simulink model "PSO_BON"  (R2019b)
settings: Solver=VariableStepAuto  StartTime=0.0  StopTime=0.2  RelTol=1e-5
undefined symbols (not defined in the file): sigbuilder_block
libraries: powerlib x164, re_lib x96, powerlib_meascontrol x9
(part 3 of 6)

== system PSO_BON/InCond1/Panel Surya/Subsystem12 ==
  In1 : Inport
  In2 : Inport  Port=2
  Diode1 : powerlib/Power Electronics/Diode  Ron=0.001  Lon=0  Vf=0.7  IC=0  UseSnubber=off  Rs=1e5*inf  Cs=inf  Measurements=off
      settings: SourceProductName=Simscape Electrical
  PV Module 5 : re_lib/Solar/PV Array  Npar=1  Nser=1  PlotType=array @ 25 deg.C & specified irradiances  S_vec="[ 1000  700  100 200]"  Temp_C_vec="[ 45 25  ]"  ModuleName=User-defined  PlotWhenSelected=off  Pm=21.837  Ncell=72  Voc=5.425  Isc=5.34  Vm=4.35  Im=5.02  beta_Voc_pc=-0.37501  alpha_Isc_pc=0.075  beta_Voc=-0.020344  alpha_Isc=0.004005  IL=5.3624  I0=3.052e-10  nI=0.12439  Rsh=79.3172  Rs=0.081018  BAL=off  Tc=1e-6  Tfilter=5e-5
      settings: SourceProductName=Simscape Electrical
  + : PMIOPort  Side=Right
  - : PMIOPort  Port=2  Side=Right
  wires:
  In1/1 -> PV Module 5/1
  In2/1 -> PV Module 5/2
  connections:
  Diode1/LConn1 -- -/RConn1 -- PV Module 5/RConn2
  +/RConn1 -- PV Module 5/RConn1 -- Diode1/RConn1

== system PSO_BON/InCond1/Panel Surya/Subsystem13 ==
  Gain{,1..3} (4 alike) : Gain  Gain=1000
  Signal Builder : Subsystem  Tag=STV Subsys  LoadFcn=sigbuilder_block('load');  StartFcn=sigbuilder_block('start');  StopFcn=sigbuilder_block('stop');  ClipboardFcn=sigbuilder_block('clipboard');  mask(Sigbuilder block){tuvar=[0:10]}
      mask help: Simulink:masks:SigbuilderBlock_MD
      mask init:
      | if ~strcmp(get_param(bdroot(gcbh),'SimulationStatus'),'stopped') tuvar = sigbuilder_block('maskInit'); end
      settings: CopyFcn=sigbuilder_block('copy');  DeleteFcn=sigbuilder_block('delete');  ModelCloseFcn=sigbuilder_block('modelClose');  PreSaveFcn=sigbuilder_block('preSave');  PauseFcn=sigbuilder_block('pause');  ContinueFcn=sigbuilder_block('continue');  NameChangeFcn=sigbuilder_block('namechange');  OpenFcn=sigbuilder_block('open',[0.75 36.75 510.75 475.5 ]);  CloseFcn=sigbuilder_block('close');
      mask Display: plot(0, 0, 100, 100,[2, 2, 32, 32, 2], [68, 8, 8, 68, 68],[32, 2], [38, 38], [32, 19, 2],[53, 60, 44], [32, 17, 17, 2],[16, 16, 31, 31]);txt = getActiveGroup(gcbh);text(2, 100, txt,'verticalAlignment', 'top');
  Out1 : Outport
  Out2 : Outport  Port=2
  Out3 : Outport  Port=3
  Out4 : Outport  Port=4
  wires:
  Gain/1 -> Out1/1
  Signal Builder/1(Signal 2) -> Gain/1
  Gain1/1 -> Out2/1
  Signal Builder/2(Signal 1) -> Gain1/1
  Gain2/1 -> Out3/1
  Signal Builder/3(Signal 3) -> Gain2/1
  Gain3/1 -> Out4/1
  Signal Builder/4(Signal 4) -> Gain3/1

== system PSO_BON/InCond1/Panel Surya/Subsystem17 ==
  In1 : Inport
  In2 : Inport  Port=2
  Diode1 : powerlib/Power Electronics/Diode  Ron=0.001  Lon=0  Vf=0.7  IC=0  UseSnubber=off  Rs=1e5*inf  Cs=inf  Measurements=off
      settings: SourceProductName=Simscape Electrical
  PV Module 5 : re_lib/Solar/PV Array  Npar=1  Nser=1  PlotType=array @ 25 deg.C & specified irradiances  S_vec="[ 1000  700  100 200]"  Temp_C_vec="[ 45 25  ]"  ModuleName=User-defined  PlotWhenSelected=off  Pm=21.837  Ncell=72  Voc=5.425  Isc=5.34  Vm=4.35  Im=5.02  beta_Voc_pc=-0.37501  alpha_Isc_pc=0.075  beta_Voc=-0.020344  alpha_Isc=0.004005  IL=5.3624  I0=3.052e-10  nI=0.12439  Rsh=79.3172  Rs=0.081018  BAL=off  Tc=1e-6  Tfilter=5e-5
      settings: SourceProductName=Simscape Electrical
  + : PMIOPort  Side=Right
  - : PMIOPort  Port=2  Side=Right
  wires:
  In2/1 -> PV Module 5/2
  In1/1 -> PV Module 5/1
  connections:
  Diode1/RConn1 -- PV Module 5/RConn1 -- +/RConn1
  PV Module 5/RConn2 -- -/RConn1 -- Diode1/LConn1

== system PSO_BON/InCond1/Panel Surya/Subsystem18 ==
  In1 : Inport
  In2 : Inport  Port=2
  Diode1 : powerlib/Power Electronics/Diode  Ron=0.001  Lon=0  Vf=0.7  IC=0  UseSnubber=off  Rs=1e5*inf  Cs=inf  Measurements=off
      settings: SourceProductName=Simscape Electrical
  PV Module 5 : re_lib/Solar/PV Array  Npar=1  Nser=1  PlotType=array @ 25 deg.C & specified irradiances  S_vec="[ 1000  700  100 200]"  Temp_C_vec="[ 45 25  ]"  ModuleName=User-defined  PlotWhenSelected=off  Pm=21.837  Ncell=72  Voc=5.425  Isc=5.34  Vm=4.35  Im=5.02  beta_Voc_pc=-0.37501  alpha_Isc_pc=0.075  beta_Voc=-0.020344  alpha_Isc=0.004005  IL=5.3624  I0=3.052e-10  nI=0.12439  Rsh=79.3172  Rs=0.081018  BAL=off  Tc=1e-6  Tfilter=5e-5
      settings: SourceProductName=Simscape Electrical
  + : PMIOPort  Side=Right
  - : PMIOPort  Port=2  Side=Right
  wires:
  In1/1 -> PV Module 5/1
  In2/1 -> PV Module 5/2
  connections:
  Diode1/LConn1 -- -/RConn1 -- PV Module 5/RConn2
  +/RConn1 -- PV Module 5/RConn1 -- Diode1/RConn1

== system PSO_BON/InCond1/Panel Surya/Subsystem19 ==
  In1 : Inport
  In2 : Inport  Port=2
  Diode1 : powerlib/Power Electronics/Diode  Ron=0.001  Lon=0  Vf=0.7  IC=0  UseSnubber=off  Rs=1e5*inf  Cs=inf  Measurements=off
      settings: SourceProductName=Simscape Electrical
  PV Module 5 : re_lib/Solar/PV Array  Npar=1  Nser=1  PlotType=array @ 25 deg.C & specified irradiances  S_vec="[ 1000  700  100 200]"  Temp_C_vec="[ 45 25  ]"  ModuleName=User-defined  PlotWhenSelected=off  Pm=21.837  Ncell=72  Voc=5.425  Isc=5.34  Vm=4.35  Im=5.02  beta_Voc_pc=-0.37501  alpha_Isc_pc=0.075  beta_Voc=-0.020344  alpha_Isc=0.004005  IL=5.3624  I0=3.052e-10  nI=0.12439  Rsh=79.3172  Rs=0.081018  BAL=off  Tc=1e-6  Tfilter=5e-5
      settings: SourceProductName=Simscape Electrical
  + : PMIOPort  Side=Right
  - : PMIOPort  Port=2  Side=Right
  wires:
  In2/1 -> PV Module 5/2
  In1/1 -> PV Module 5/1
  connections:
  Diode1/RConn1 -- PV Module 5/RConn1 -- +/RConn1
  PV Module 5/RConn2 -- -/RConn1 -- Diode1/LConn1

== system PSO_BON/InCond1/Panel Surya/Subsystem2 ==
  In1 : Inport
  In2 : Inport  Port=2
  Diode1 : powerlib/Power Electronics/Diode  Ron=0.001  Lon=0  Vf=0.7  IC=0  UseSnubber=off  Rs=1e5*inf  Cs=inf  Measurements=off
      settings: SourceProductName=Simscape Electrical
  PV Module 5 : re_lib/Solar/PV Array  Npar=1  Nser=1  PlotType=one module @ 25 deg.C & specified irradiances  S_vec="[ 1000  800  100 200]"  Temp_C_vec="[ 45 25  ]"  ModuleName=SunPower SPR-315E-WHT-D  PlotWhenSelected=off  Pm=315.072  Ncell=96  Voc=64.6  Isc=6.14  Vm=54.7  Im=5.76  beta_Voc_pc=-0.27269  alpha_Isc_pc=0.061694  beta_Voc=-0.17616  alpha_Isc=0.003788  IL=6.1461  I0=6.5043e-12  nI=0.9507  Rsh=430.0559  Rs=0.43042  BAL=off  Tc=1e-6  Tfilter=5e-5
      settings: SourceProductName=Simscape Electrical
  + : PMIOPort  Side=Right
  - : PMIOPort  Port=2  Side=Right
  wires:
  In1/1 -> PV Module 5/1
  In2/1 -> PV Module 5/2
  connections:
  Diode1/LConn1 -- -/RConn1 -- PV Module 5/RConn2
  +/RConn1 -- PV Module 5/RConn1 -- Diode1/RConn1

== system PSO_BON/InCond1/Panel Surya/Subsystem3 ==
  In1 : Inport
  In2 : Inport  Port=2
  Diode1 : powerlib/Power Electronics/Diode  Ron=0.001  Lon=0  Vf=0.7  IC=0  UseSnubber=off  Rs=1e5*inf  Cs=inf  Measurements=off
      settings: SourceProductName=Simscape Electrical
  PV Module 5 : re_lib/Solar/PV Array  Npar=1  Nser=1  PlotType=one module @ 25 deg.C & specified irradiances  S_vec="[ 1000  800  100 200]"  Temp_C_vec="[ 45 25  ]"  ModuleName=SunPower SPR-315E-WHT-D  PlotWhenSelected=off  Pm=315.072  Ncell=96  Voc=64.6  Isc=6.14  Vm=54.7  Im=5.76  beta_Voc_pc=-0.27269  alpha_Isc_pc=0.061694  beta_Voc=-0.17616  alpha_Isc=0.003788  IL=6.1461  I0=6.5043e-12  nI=0.9507  Rsh=430.0559  Rs=0.43042  BAL=off  Tc=1e-6  Tfilter=5e-5
      settings: SourceProductName=Simscape Electrical
  + : PMIOPort  Side=Right
  - : PMIOPort  Port=2  Side=Right
  wires:
  In2/1 -> PV Module 5/2
  In1/1 -> PV Module 5/1
  connections:
  Diode1/RConn1 -- PV Module 5/RConn1 -- +/RConn1
  PV Module 5/RConn2 -- -/RConn1 -- Diode1/LConn1

== system PSO_BON/InCond1/Panel Surya/Subsystem4 ==
  In1 : Inport
  In2 : Inport  Port=2
  Diode1 : powerlib/Power Electronics/Diode  Ron=0.001  Lon=0  Vf=0.7  IC=0  UseSnubber=off  Rs=1e5*inf  Cs=inf  Measurements=off
      settings: SourceProductName=Simscape Electrical
  PV Module 5 : re_lib/Solar/PV Array  Npar=1  Nser=1  PlotType=one module @ 25 deg.C & specified irradiances  S_vec="[ 1000  800  100 200]"  Temp_C_vec="[ 45 25  ]"  ModuleName=SunPower SPR-315E-WHT-D  PlotWhenSelected=off  Pm=315.072  Ncell=96  Voc=64.6  Isc=6.14  Vm=54.7  Im=5.76  beta_Voc_pc=-0.27269  alpha_Isc_pc=0.061694  beta_Voc=-0.17616  alpha_Isc=0.003788  IL=6.1461  I0=6.5043e-12  nI=0.9507  Rsh=430.0559  Rs=0.43042  BAL=off  Tc=1e-6  Tfilter=1.25e-5
      settings: SourceProductName=Simscape Electrical
  + : PMIOPort  Side=Right
  - : PMIOPort  Port=2  Side=Right
  wires:
  In2/1 -> PV Module 5/2
  In1/1 -> PV Module 5/1
  connections:
  Diode1/RConn1 -- PV Module 5/RConn1 -- +/RConn1
  PV Module 5/RConn2 -- -/RConn1 -- Diode1/LConn1

== system PSO_BON/InCond1/Panel Surya/Subsystem5 ==
  In1 : Inport
  In2 : Inport  Port=2
  Diode1 : powerlib/Power Electronics/Diode  Ron=0.001  Lon=0  Vf=0.7  IC=0  UseSnubber=off  Rs=1e5*inf  Cs=inf  Measurements=off
      settings: SourceProductName=Simscape Electrical
  PV Module 5 : re_lib/Solar/PV Array  Npar=1  Nser=1  PlotType=one module @ 25 deg.C & specified irradiances  S_vec="[ 1000  800  100 200]"  Temp_C_vec="[ 45 25  ]"  ModuleName=SunPower SPR-315E-WHT-D  PlotWhenSelected=off  Pm=315.072  Ncell=96  Voc=64.6  Isc=6.14  Vm=54.7  Im=5.76  beta_Voc_pc=-0.27269  alpha_Isc_pc=0.061694  beta_Voc=-0.17616  alpha_Isc=0.003788  IL=6.1461  I0=6.5043e-12  nI=0.9507  Rsh=430.0559  Rs=0.43042  BAL=off  Tc=1e-6  Tfilter=1.25e-5
      settings: SourceProductName=Simscape Electrical
  + : PMIOPort  Side=Right
  - : PMIOPort  Port=2  Side=Right
  wires:
  In1/1 -> PV Module 5/1
  In2/1 -> PV Module 5/2
  connections:
  Diode1/LConn1 -- -/RConn1 -- PV Module 5/RConn2
  +/RConn1 -- PV Module 5/RConn1 -- Diode1/RConn1

== system PSO_BON/InCond1/Panel Surya/Subsystem6 ==
  In1 : Inport
  In2 : Inport  Port=2
  Diode1 : powerlib/Power Electronics/Diode  Ron=0.001  Lon=0  Vf=0.7  IC=0  UseSnubber=off  Rs=1e5*inf  Cs=inf  Measurements=off
      settings: SourceProductName=Simscape Electrical
  PV Module 5 : re_lib/Solar/PV Array  Npar=1  Nser=1  PlotType=one module @ 25 deg.C & specified irradiances  S_vec="[ 1000  800  100 200]"  Temp_C_vec="[ 45 25  ]"  ModuleName=SunPower SPR-315E-WHT-D  PlotWhenSelected=off  Pm=315.072  Ncell=96  Voc=64.6  Isc=6.14  Vm=54.7  Im=5.76  beta_Voc_pc=-0.27269  alpha_Isc_pc=0.061694  beta_Voc=-0.17616  alpha_Isc=0.003788  IL=6.1461  I0=6.5043e-12  nI=0.9507  Rsh=430.0559  Rs=0.43042  BAL=off  Tc=1e-6  Tfilter=1.25e-5
      settings: SourceProductName=Simscape Electrical
  + : PMIOPort  Side=Right
  - : PMIOPort  Port=2  Side=Right
  wires:
  In2/1 -> PV Module 5/2
  In1/1 -> PV Module 5/1
  connections:
  Diode1/RConn1 -- PV Module 5/RConn1 -- +/RConn1
  PV Module 5/RConn2 -- -/RConn1 -- Diode1/LConn1

== system PSO_BON/InCond1/Panel Surya/Subsystem7 ==
  In1 : Inport
  In2 : Inport  Port=2
  Diode1 : powerlib/Power Electronics/Diode  Ron=0.001  Lon=0  Vf=0.7  IC=0  UseSnubber=off  Rs=1e5*inf  Cs=inf  Measurements=off
      settings: SourceProductName=Simscape Electrical
  PV Module 5 : re_lib/Solar/PV Array  Npar=1  Nser=1  PlotType=one module @ 25 deg.C & specified irradiances  S_vec="[ 1000  800  100 200]"  Temp_C_vec="[ 45 25  ]"  ModuleName=SunPower SPR-315E-WHT-D  PlotWhenSelected=off  Pm=315.072  Ncell=96  Voc=64.6  Isc=6.14  Vm=54.7  Im=5.76  beta_Voc_pc=-0.27269  alpha_Isc_pc=0.061694  beta_Voc=-0.17616  alpha_Isc=0.003788  IL=6.1461  I0=6.5043e-12  nI=0.9507  Rsh=430.0559  Rs=0.43042  BAL=off  Tc=1e-6  Tfilter=1.25e-5
      settings: SourceProductName=Simscape Electrical
  + : PMIOPort  Side=Right
  - : PMIOPort  Port=2  Side=Right
  wires:
  In1/1 -> PV Module 5/1
  In2/1 -> PV Module 5/2
  connections:
  Diode1/LConn1 -- -/RConn1 -- PV Module 5/RConn2
  +/RConn1 -- PV Module 5/RConn1 -- Diode1/RConn1

== system PSO_BON/P&O/Panel Surya/Subsystem ==
  In1 : Inport
  In2 : Inport  Port=2
  Diode1 : powerlib/Power Electronics/Diode  Ron=0.001  Lon=0  Vf=0.7  IC=0  UseSnubber=off  Rs=1e5*inf  Cs=inf  Measurements=off
      settings: SourceProductName=Simscape Electrical
  PV Module 5 : re_lib/Solar/PV Array  Npar=2  Nser=1  PlotType=one module @ 25 deg.C & specified irradiances  S_vec="[ 1000  800  100 200]"  Temp_C_vec="[ 45 25  ]"  ModuleName=SunPower SPR-315E-WHT-D  PlotWhenSelected=off  Pm=315.072  Ncell=96  Voc=64.6  Isc=6.14  Vm=54.7  Im=5.76  beta_Voc_pc=-0.27269  alpha_Isc_pc=0.061694  beta_Voc=-0.17616  alpha_Isc=0.003788  IL=6.1461  I0=6.5043e-12  nI=0.9507  Rsh=430.0559  Rs=0.43042  BAL=off  Tc=1e-6  Tfilter=5e-5
      settings: SourceProductName=Simscape Electrical
  + : PMIOPort  Side=Right
  - : PMIOPort  Port=2  Side=Right
  wires:
  In2/1 -> PV Module 5/2
  In1/1 -> PV Module 5/1
  connections:
  Diode1/RConn1 -- PV Module 5/RConn1 -- +/RConn1
  PV Module 5/RConn2 -- -/RConn1 -- Diode1/LConn1

== system PSO_BON/P&O/Panel Surya/Subsystem1 ==
  In1 : Inport
  In2 : Inport  Port=2
  Diode1 : powerlib/Power Electronics/Diode  Ron=0.001  Lon=0  Vf=0.7  IC=0  UseSnubber=off  Rs=1e5*inf  Cs=inf  Measurements=off
      settings: SourceProductName=Simscape Electrical
  PV Module 5 : re_lib/Solar/PV Array  Npar=2  Nser=1  PlotType=one module @ 25 deg.C & specified irradiances  S_vec="[ 1000  800  100 200]"  Temp_C_vec="[ 45 25  ]"  ModuleName=SunPower SPR-315E-WHT-D  PlotWhenSelected=off  Pm=315.072  Ncell=96  Voc=64.6  Isc=6.14  Vm=54.7  Im=5.76  beta_Voc_pc=-0.27269  alpha_Isc_pc=0.061694  beta_Voc=-0.17616  alpha_Isc=0.003788  IL=6.1461  I0=6.5043e-12  nI=0.9507  Rsh=430.0559  Rs=0.43042  BAL=off  Tc=1e-6  Tfilter=5e-5
      settings: SourceProductName=Simscape Electrical
  + : PMIOPort  Side=Right
  - : PMIOPort  Port=2  Side=Right
  wires:
  In1/1 -> PV Module 5/1
  In2/1 -> PV Module 5/2
  connections:
  Diode1/LConn1 -- -/RConn1 -- PV Module 5/RConn2
  +/RConn1 -- PV Module 5/RConn1 -- Diode1/RConn1

== system PSO_BON/P&O/Panel Surya/Subsystem2 ==
  In1 : Inport
  In2 : Inport  Port=2
  Diode1 : powerlib/Power Electronics/Diode  Ron=0.001  Lon=0  Vf=0.7  IC=0  UseSnubber=off  Rs=1e5*inf  Cs=inf  Measurements=off
      settings: SourceProductName=Simscape Electrical
  PV Module 5 : re_lib/Solar/PV Array  Npar=2  Nser=1  PlotType=one module @ 25 deg.C & specified irradiances  S_vec="[ 1000  800  100 200]"  Temp_C_vec="[ 45 25  ]"  ModuleName=SunPower SPR-315E-WHT-D  PlotWhenSelected=off  Pm=315.072  Ncell=96  Voc=64.6  Isc=6.14  Vm=54.7  Im=5.76  beta_Voc_pc=-0.27269  alpha_Isc_pc=0.061694  beta_Voc=-0.17616  alpha_Isc=0.003788  IL=6.1461  I0=6.5043e-12  nI=0.9507  Rsh=430.0559  Rs=0.43042  BAL=off  Tc=1e-6  Tfilter=5e-5
      settings: SourceProductName=Simscape Electrical
  + : PMIOPort  Side=Right
  - : PMIOPort  Port=2  Side=Right
  wires:
  In2/1 -> PV Module 5/2
  In1/1 -> PV Module 5/1
  connections:
  Diode1/RConn1 -- PV Module 5/RConn1 -- +/RConn1
  PV Module 5/RConn2 -- -/RConn1 -- Diode1/LConn1

== system PSO_BON/P&O/Panel Surya/Subsystem3 ==
  In1 : Inport
  In2 : Inport  Port=2
  Diode1 : powerlib/Power Electronics/Diode  Ron=0.001  Lon=0  Vf=0.7  IC=0  UseSnubber=off  Rs=1e5*inf  Cs=inf  Measurements=off
      settings: SourceProductName=Simscape Electrical
  PV Module 5 : re_lib/Solar/PV Array  Npar=2  Nser=1  PlotType=one module @ 25 deg.C & specified irradiances  S_vec="[ 1000  800  100 200]"  Temp_C_vec="[ 45 25  ]"  ModuleName=SunPower SPR-315E-WHT-D  PlotWhenSelected=off  Pm=315.072  Ncell=96  Voc=64.6  Isc=6.14  Vm=54.7  Im=5.76  beta_Voc_pc=-0.27269  alpha_Isc_pc=0.061694  beta_Voc=-0.17616  alpha_Isc=0.003788  IL=6.1461  I0=6.5043e-12  nI=0.9507  Rsh=430.0559  Rs=0.43042  BAL=off  Tc=1e-6  Tfilter=5e-5
      settings: SourceProductName=Simscape Electrical
  + : PMIOPort  Side=Right
  - : PMIOPort  Port=2  Side=Right
  wires:
  In1/1 -> PV Module 5/1
  In2/1 -> PV Module 5/2
  connections:
  Diode1/LConn1 -- -/RConn1 -- PV Module 5/RConn2
  +/RConn1 -- PV Module 5/RConn1 -- Diode1/RConn1

== system PSO_BON/P&O/Panel Surya/Subsystem4 ==
  In1 : Inport
  In2 : Inport  Port=2
  Diode1 : powerlib/Power Electronics/Diode  Ron=0.001  Lon=0  Vf=0.7  IC=0  UseSnubber=off  Rs=1e5*inf  Cs=inf  Measurements=off
      settings: SourceProductName=Simscape Electrical
  PV Module 5 : re_lib/Solar/PV Array  Npar=1  Nser=1  PlotType=one module @ 25 deg.C & specified irradiances  S_vec="[ 1000  800  100 200]"  Temp_C_vec="[ 45 25  ]"  ModuleName=SunPower SPR-315E-WHT-D  PlotWhenSelected=off  Pm=315.072  Ncell=96  Voc=64.6  Isc=6.14  Vm=54.7  Im=5.76  beta_Voc_pc=-0.27269  alpha_Isc_pc=0.061694  beta_Voc=-0.17616  alpha_Isc=0.003788  IL=6.1461  I0=6.5043e-12  nI=0.9507  Rsh=430.0559  Rs=0.43042  BAL=off  Tc=1e-6  Tfilter=5e-5
      settings: SourceProductName=Simscape Electrical
  + : PMIOPort  Side=Right
  - : PMIOPort  Port=2  Side=Right
  wires:
  In1/1 -> PV Module 5/1
  In2/1 -> PV Module 5/2
  connections:
  Diode1/LConn1 -- -/RConn1 -- PV Module 5/RConn2
  +/RConn1 -- PV Module 5/RConn1 -- Diode1/RConn1

== system PSO_BON/P&O/Panel Surya/Subsystem5 ==
  In1 : Inport
  In2 : Inport  Port=2
  Diode1 : powerlib/Power Electronics/Diode  Ron=0.001  Lon=0  Vf=0.7  IC=0  UseSnubber=off  Rs=1e5*inf  Cs=inf  Measurements=off
      settings: SourceProductName=Simscape Electrical
  PV Module 5 : re_lib/Solar/PV Array  Npar=1  Nser=1  PlotType=one module @ 25 deg.C & specified irradiances  S_vec="[ 1000  800  100 200]"  Temp_C_vec="[ 45 25  ]"  ModuleName=SunPower SPR-315E-WHT-D  PlotWhenSelected=off  Pm=315.072  Ncell=96  Voc=64.6  Isc=6.14  Vm=54.7  Im=5.76  beta_Voc_pc=-0.27269  alpha_Isc_pc=0.061694  beta_Voc=-0.17616  alpha_Isc=0.003788  IL=6.1461  I0=6.5043e-12  nI=0.9507  Rsh=430.0559  Rs=0.43042  BAL=off  Tc=1e-6  Tfilter=5e-5
      settings: SourceProductName=Simscape Electrical
  + : PMIOPort  Side=Right
  - : PMIOPort  Port=2  Side=Right
  wires:
  In2/1 -> PV Module 5/2
  In1/1 -> PV Module 5/1
  connections:
  Diode1/RConn1 -- PV Module 5/RConn1 -- +/RConn1
  PV Module 5/RConn2 -- -/RConn1 -- Diode1/LConn1

== system PSO_BON/P&O/Panel Surya/Subsystem6 ==
  In1 : Inport
  In2 : Inport  Port=2
  Diode1 : powerlib/Power Electronics/Diode  Ron=0.001  Lon=0  Vf=0.7  IC=0  UseSnubber=off  Rs=1e5*inf  Cs=inf  Measurements=off
      settings: SourceProductName=Simscape Electrical
  PV Module 5 : re_lib/Solar/PV Array  Npar=1  Nser=1  PlotType=one module @ 25 deg.C & specified irradiances  S_vec="[ 1000  800  100 200]"  Temp_C_vec="[ 45 25  ]"  ModuleName=SunPower SPR-315E-WHT-D  PlotWhenSelected=off  Pm=315.072  Ncell=96  Voc=64.6  Isc=6.14  Vm=54.7  Im=5.76  beta_Voc_pc=-0.27269  alpha_Isc_pc=0.061694  beta_Voc=-0.17616  alpha_Isc=0.003788  IL=6.1461  I0=6.5043e-12  nI=0.9507  Rsh=430.0559  Rs=0.43042  BAL=off  Tc=1e-6  Tfilter=5e-5
      settings: SourceProductName=Simscape Electrical
  + : PMIOPort  Side=Right
  - : PMIOPort  Port=2  Side=Right
  wires:
  In1/1 -> PV Module 5/1
  In2/1 -> PV Module 5/2
  connections:
  Diode1/LConn1 -- -/RConn1 -- PV Module 5/RConn2
  +/RConn1 -- PV Module 5/RConn1 -- Diode1/RConn1

== system PSO_BON/P&O/Panel Surya/Subsystem7 ==
  In1 : Inport
  In2 : Inport  Port=2
  Diode1 : powerlib/Power Electronics/Diode  Ron=0.001  Lon=0  Vf=0.7  IC=0  UseSnubber=off  Rs=1e5*inf  Cs=inf  Measurements=off
      settings: SourceProductName=Simscape Electrical
  PV Module 5 : re_lib/Solar/PV Array  Npar=1  Nser=1  PlotType=one module @ 25 deg.C & specified irradiances  S_vec="[ 1000  800  100 200]"  Temp_C_vec="[ 45 25  ]"  ModuleName=SunPower SPR-315E-WHT-D  PlotWhenSelected=off  Pm=315.072  Ncell=96  Voc=64.6  Isc=6.14  Vm=54.7  Im=5.76  beta_Voc_pc=-0.27269  alpha_Isc_pc=0.061694  beta_Voc=-0.17616  alpha_Isc=0.003788  IL=6.1461  I0=6.5043e-12  nI=0.9507  Rsh=430.0559  Rs=0.43042  BAL=off  Tc=1e-6  Tfilter=5e-5
      settings: SourceProductName=Simscape Electrical
  + : PMIOPort  Side=Right
  - : PMIOPort  Port=2  Side=Right
  wires:
  In2/1 -> PV Module 5/2
  In1/1 -> PV Module 5/1
  connections:
  Diode1/RConn1 -- PV Module 5/RConn1 -- +/RConn1
  PV Module 5/RConn2 -- -/RConn1 -- Diode1/LConn1

== system PSO_BON/Phasor PSO1/Panel Surya/Subsystem ==
  In1 : Inport
  In2 : Inport  Port=2
  Diode1 : powerlib/Power Electronics/Diode  Ron=0.001  Lon=0  Vf=0.7  IC=0  UseSnubber=off  Rs=1e5*inf  Cs=inf  Measurements=off
      settings: SourceProductName=Simscape Electrical
  PV Module 5 : re_lib/Solar/PV Array  Npar=1  Nser=1  PlotType=one module @ 25 deg.C & specified irradiances  S_vec="[ 1000  800  100 200]"  Temp_C_vec="[ 45 25  ]"  ModuleName=SunPower SPR-315E-WHT-D  PlotWhenSelected=off  Pm=315.072  Ncell=96  Voc=64.6  Isc=6.14  Vm=54.7  Im=5.76  beta_Voc_pc=-0.27269  alpha_Isc_pc=0.061694  beta_Voc=-0.17616  alpha_Isc=0.003788  IL=6.1461  I0=6.5043e-12  nI=0.9507  Rsh=430.0559  Rs=0.43042  BAL=off  Tc=1e-6  Tfilter=5e-5
      settings: SourceProductName=Simscape Electrical
  + : PMIOPort  Side=Right
  - : PMIOPort  Port=2  Side=Right
  wires:
  In1/1 -> PV Module 5/1
  In2/1 -> PV Module 5/2
  connections:
  Diode1/LConn1 -- -/RConn1 -- PV Module 5/RConn2
  +/RConn1 -- PV Module 5/RConn1 -- Diode1/RConn1

== system PSO_BON/Phasor PSO1/Panel Surya/Subsystem1 ==
  In1 : Inport
  In2 : Inport  Port=2
  Diode1 : powerlib/Power Electronics/Diode  Ron=0.001  Lon=0  Vf=0.7  IC=0  UseSnubber=off  Rs=1e5*inf  Cs=inf  Measurements=off
      settings: SourceProductName=Simscape Electrical
  PV Module 5 : re_lib/Solar/PV Array  Npar=1  Nser=1  PlotType=one module @ 25 deg.C & specified irradiances  S_vec="[ 1000  800  100 200]"  Temp_C_vec="[ 45 25  ]"  ModuleName=SunPower SPR-315E-WHT-D  PlotWhenSelected=off  Pm=315.072  Ncell=96  Voc=64.6  Isc=6.14  Vm=54.7  Im=5.76  beta_Voc_pc=-0.27269  alpha_Isc_pc=0.061694  beta_Voc=-0.17616  alpha_Isc=0.003788  IL=6.1461  I0=6.5043e-12  nI=0.9507  Rsh=430.0559  Rs=0.43042  BAL=off  Tc=1e-6  Tfilter=5e-5
      settings: SourceProductName=Simscape Electrical
  + : PMIOPort  Side=Right
  - : PMIOPort  Port=2  Side=Right
  wires:
  In2/1 -> PV Module 5/2
  In1/1 -> PV Module 5/1
  connections:
  Diode1/RConn1 -- PV Module 5/RConn1 -- +/RConn1
  PV Module 5/RConn2 -- -/RConn1 -- Diode1/LConn1

== system PSO_BON/Phasor PSO1/Panel Surya/Subsystem10 ==
  Gain{,1..3} (4 alike) : Gain  Gain=1000
  Signal Builder : Subsystem  Tag=STV Subsys  LoadFcn=sigbuilder_block('load');  StartFcn=sigbuilder_block('start');  StopFcn=sigbuilder_block('stop');  ClipboardFcn=sigbuilder_block('clipboard');  mask(Sigbuilder block){tuvar=[0:10]}
      mask help: Simulink:masks:SigbuilderBlock_MD
      mask init:
      | if ~strcmp(get_param(bdroot(gcbh),'SimulationStatus'),'stopped') tuvar = sigbuilder_block('maskInit'); end
      settings: CopyFcn=sigbuilder_block('copy');  DeleteFcn=sigbuilder_block('delete');  ModelCloseFcn=sigbuilder_block('modelClose');  PreSaveFcn=sigbuilder_block('preSave');  PauseFcn=sigbuilder_block('pause');  ContinueFcn=sigbuilder_block('continue');  NameChangeFcn=sigbuilder_block('namechange');  OpenFcn=sigbuilder_block('open',[0.75 36.75 510.75 475.5 ]);  CloseFcn=sigbuilder_block('close');
      mask Display: plot(0, 0, 100, 100,[2, 2, 32, 32, 2], [68, 8, 8, 68, 68],[32, 2], [38, 38], [32, 19, 2],[53, 60, 44], [32, 17, 17, 2],[16, 16, 31, 31]);txt = getActiveGroup(gcbh);text(2, 100, txt,'verticalAlignment', 'top');
  Out1 : Outport
  Out2 : Outport  Port=2
  Out3 : Outport  Port=3
  Out4 : Outport  Port=4
  wires:
  Signal Builder/4(Signal 4) -> Gain3/1
  Gain3/1 -> Out4/1
  Signal Builder/3(Signal 3) -> Gain2/1
  Gain2/1 -> Out3/1
  Signal Builder/2(Signal 1) -> Gain1/1
  Gain1/1 -> Out2/1
  Signal Builder/1(Signal 2) -> Gain/1
  Gain/1 -> Out1/1

== system PSO_BON/Phasor PSO1/Panel Surya/Subsystem11 ==
  Gain{,1..3} (4 alike) : Gain  Gain=1000
  Signal Builder : Subsystem  Tag=STV Subsys  LoadFcn=sigbuilder_block('load');  StartFcn=sigbuilder_block('start');  StopFcn=sigbuilder_block('stop');  ClipboardFcn=sigbuilder_block('clipboard');  mask(Sigbuilder block){tuvar=[0:10]}
      mask help: Simulink:masks:SigbuilderBlock_MD
      mask init:
      | if ~strcmp(get_param(bdroot(gcbh),'SimulationStatus'),'stopped') tuvar = sigbuilder_block('maskInit'); end
      settings: CopyFcn=sigbuilder_block('copy');  DeleteFcn=sigbuilder_block('delete');  ModelCloseFcn=sigbuilder_block('modelClose');  PreSaveFcn=sigbuilder_block('preSave');  PauseFcn=sigbuilder_block('pause');  ContinueFcn=sigbuilder_block('continue');  NameChangeFcn=sigbuilder_block('namechange');  OpenFcn=sigbuilder_block('open',[0.75 36.75 510.75 475.5 ]);  CloseFcn=sigbuilder_block('close');
      mask Display: plot(0, 0, 100, 100,[2, 2, 32, 32, 2], [68, 8, 8, 68, 68],[32, 2], [38, 38], [32, 19, 2],[53, 60, 44], [32, 17, 17, 2],[16, 16, 31, 31]);txt = getActiveGroup(gcbh);text(2, 100, txt,'verticalAlignment', 'top');
  Out1 : Outport
  Out2 : Outport  Port=2
  Out3 : Outport  Port=3
  Out4 : Outport  Port=4
  wires:
  Gain/1 -> Out1/1
  Signal Builder/1(Signal 2) -> Gain/1
  Gain1/1 -> Out2/1
  Signal Builder/2(Signal 1) -> Gain1/1
  Gain2/1 -> Out3/1
  Signal Builder/3(Signal 3) -> Gain2/1
  Gain3/1 -> Out4/1
  Signal Builder/4(Signal 4) -> Gain3/1

== system PSO_BON/Phasor PSO1/Panel Surya/Subsystem12 ==
  In1 : Inport
  In2 : Inport  Port=2
  Diode1 : powerlib/Power Electronics/Diode  Ron=0.001  Lon=0  Vf=0.7  IC=0  UseSnubber=off  Rs=1e5*inf  Cs=inf  Measurements=off
      settings: SourceProductName=Simscape Electrical
  PV Module 5 : re_lib/Solar/PV Array  Npar=1  Nser=1  PlotType=array @ 25 deg.C & specified irradiances  S_vec="[ 1000  700  100 200]"  Temp_C_vec="[ 45 25  ]"  ModuleName=User-defined  PlotWhenSelected=off  Pm=21.837  Ncell=72  Voc=5.425  Isc=5.34  Vm=4.35  Im=5.02  beta_Voc_pc=-0.37501  alpha_Isc_pc=0.075  beta_Voc=-0.020344  alpha_Isc=0.004005  IL=5.3624  I0=3.052e-10  nI=0.12439  Rsh=79.3172  Rs=0.081018  BAL=off  Tc=1e-6  Tfilter=5e-5
      settings: SourceProductName=Simscape Electrical
  + : PMIOPort  Side=Right
  - : PMIOPort  Port=2  Side=Right
  wires:
  In1/1 -> PV Module 5/1
  In2/1 -> PV Module 5/2
  connections:
  Diode1/LConn1 -- -/RConn1 -- PV Module 5/RConn2
  +/RConn1 -- PV Module 5/RConn1 -- Diode1/RConn1

== system PSO_BON/Phasor PSO1/Panel Surya/Subsystem13 ==
  Gain{,1..3} (4 alike) : Gain  Gain=1000
  Signal Builder : Subsystem  Tag=STV Subsys  LoadFcn=sigbuilder_block('load');  StartFcn=sigbuilder_block('start');  StopFcn=sigbuilder_block('stop');  ClipboardFcn=sigbuilder_block('clipboard');  mask(Sigbuilder block){tuvar=[0:10]}
      mask help: Simulink:masks:SigbuilderBlock_MD
      mask init:
      | if ~strcmp(get_param(bdroot(gcbh),'SimulationStatus'),'stopped') tuvar = sigbuilder_block('maskInit'); end
      settings: CopyFcn=sigbuilder_block('copy');  DeleteFcn=sigbuilder_block('delete');  ModelCloseFcn=sigbuilder_block('modelClose');  PreSaveFcn=sigbuilder_block('preSave');  PauseFcn=sigbuilder_block('pause');  ContinueFcn=sigbuilder_block('continue');  NameChangeFcn=sigbuilder_block('namechange');  OpenFcn=sigbuilder_block('open',[0 36 1440 716.25 ]);  CloseFcn=sigbuilder_block('close');
      mask Display: plot(0, 0, 100, 100,[2, 2, 32, 32, 2], [68, 8, 8, 68, 68],[32, 2], [38, 38], [32, 19, 2],[53, 60, 44], [32, 17, 17, 2],[16, 16, 31, 31]);txt = getActiveGroup(gcbh);text(2, 100, txt,'verticalAlignment', 'top');
  Out1 : Outport
  Out2 : Outport  Port=2
  Out3 : Outport  Port=3
  Out4 : Outport  Port=4
  wires:
  Gain/1 -> Out1/1
  Signal Builder/1(Signal 2) -> Gain/1
  Signal Builder/3(Signal 3) -> Gain2/1
  Signal Builder/2(Signal 1) -> Gain1/1
  Signal Builder/4(Signal 4) -> Gain3/1
  Gain1/1 -> Out2/1
  Gain2/1 -> Out3/1
  Gain3/1 -> Out4/1

== system PSO_BON/Phasor PSO1/Panel Surya/Subsystem14 ==
  Gain{,1..3} (4 alike) : Gain  Gain=1000
  Signal Builder : Subsystem  Tag=STV Subsys  LoadFcn=sigbuilder_block('load');  StartFcn=sigbuilder_block('start');  StopFcn=sigbuilder_block('stop');  ClipboardFcn=sigbuilder_block('clipboard');  mask(Sigbuilder block){tuvar=[0:10]}
      mask help: Simulink:masks:SigbuilderBlock_MD
      mask init:
      | if ~strcmp(get_param(bdroot(gcbh),'SimulationStatus'),'stopped') tuvar = sigbuilder_block('maskInit'); end
      settings: CopyFcn=sigbuilder_block('copy');  DeleteFcn=sigbuilder_block('delete');  ModelCloseFcn=sigbuilder_block('modelClose');  PreSaveFcn=sigbuilder_block('preSave');  PauseFcn=sigbuilder_block('pause');  ContinueFcn=sigbuilder_block('continue');  NameChangeFcn=sigbuilder_block('namechange');  OpenFcn=sigbuilder_block('open',[159 193.5 551.25 399.75 ]);  CloseFcn=sigbuilder_block('close');
      mask Display: plot(0, 0, 100, 100,[2, 2, 32, 32, 2], [68, 8, 8, 68, 68],[32, 2], [38, 38], [32, 19, 2],[53, 60, 44], [32, 17, 17, 2],[16, 16, 31, 31]);txt = getActiveGroup(gcbh);text(2, 100, txt,'verticalAlignment', 'top');
  Out1 : Outport
  Out2 : Outport  Port=2
  Out3 : Outport  Port=3
  Out4 : Outport  Port=4
  wires:
  Signal Builder/1(Signal 2) -> Gain/1
  Gain/1 -> Out1/1
  Signal Builder/2(Signal 1) -> Gain1/1
  Signal Builder/3(Signal 3) -> Gain2/1
  Signal Builder/4(Signal 4) -> Gain3/1
  Gain1/1 -> Out2/1
  Gain2/1 -> Out3/1
  Gain3/1 -> Out4/1

== system PSO_BON/Phasor PSO1/Panel Surya/Subsystem17 ==
  In1 : Inport
  In2 : Inport  Port=2
  Diode1 : powerlib/Power Electronics/Diode  Ron=0.001  Lon=0  Vf=0.7  IC=0  UseSnubber=off  Rs=1e5*inf  Cs=inf  Measurements=off
      settings: SourceProductName=Simscape Electrical
  PV Module 5 : re_lib/Solar/PV Array  Npar=1  Nser=1  PlotType=array @ 25 deg.C & specified irradiances  S_vec="[ 1000  700  100 200]"  Temp_C_vec="[ 45 25  ]"  ModuleName=User-defined  PlotWhenSelected=off  Pm=21.837  Ncell=72  Voc=5.425  Isc=5.34  Vm=4.35  Im=5.02  beta_Voc_pc=-0.37501  alpha_Isc_pc=0.075  beta_Voc=-0.020344  alpha_Isc=0.004005  IL=5.3624  I0=3.052e-10  nI=0.12439  Rsh=79.3172  Rs=0.081018  BAL=off  Tc=1e-6  Tfilter=5e-5
      settings: SourceProductName=Simscape Electrical
  + : PMIOPort  Side=Right
  - : PMIOPort  Port=2  Side=Right
  wires:
  In2/1 -> PV Module 5/2
  In1/1 -> PV Module 5/1
  connections:
  Diode1/RConn1 -- PV Module 5/RConn1 -- +/RConn1
  PV Module 5/RConn2 -- -/RConn1 -- Diode1/LConn1

== system PSO_BON/Phasor PSO1/Panel Surya/Subsystem18 ==
  In1 : Inport
  In2 : Inport  Port=2
  Diode1 : powerlib/Power Electronics/Diode  Ron=0.001  Lon=0  Vf=0.7  IC=0  UseSnubber=off  Rs=1e5*inf  Cs=inf  Measurements=off
      settings: SourceProductName=Simscape Electrical
  PV Module 5 : re_lib/Solar/PV Array  Npar=1  Nser=1  PlotType=array @ 25 deg.C & specified irradiances  S_vec="[ 1000  700  100 200]"  Temp_C_vec="[ 45 25  ]"  ModuleName=User-defined  PlotWhenSelected=off  Pm=21.837  Ncell=72  Voc=5.425  Isc=5.34  Vm=4.35  Im=5.02  beta_Voc_pc=-0.37501  alpha_Isc_pc=0.075  beta_Voc=-0.020344  alpha_Isc=0.004005  IL=5.3624  I0=3.052e-10  nI=0.12439  Rsh=79.3172  Rs=0.081018  BAL=off  Tc=1e-6  Tfilter=5e-5
      settings: SourceProductName=Simscape Electrical
  + : PMIOPort  Side=Right
  - : PMIOPort  Port=2  Side=Right
  wires:
  In1/1 -> PV Module 5/1
  In2/1 -> PV Module 5/2
  connections:
  Diode1/LConn1 -- -/RConn1 -- PV Module 5/RConn2
  +/RConn1 -- PV Module 5/RConn1 -- Diode1/RConn1

== system PSO_BON/Phasor PSO1/Panel Surya/Subsystem19 ==
  In1 : Inport
  In2 : Inport  Port=2
  Diode1 : powerlib/Power Electronics/Diode  Ron=0.001  Lon=0  Vf=0.7  IC=0  UseSnubber=off  Rs=1e5*inf  Cs=inf  Measurements=off
      settings: SourceProductName=Simscape Electrical
  PV Module 5 : re_lib/Solar/PV Array  Npar=1  Nser=1  PlotType=array @ 25 deg.C & specified irradiances  S_vec="[ 1000  700  100 200]"  Temp_C_vec="[ 45 25  ]"  ModuleName=User-defined  PlotWhenSelected=off  Pm=21.837  Ncell=72  Voc=5.425  Isc=5.34  Vm=4.35  Im=5.02  beta_Voc_pc=-0.37501  alpha_Isc_pc=0.075  beta_Voc=-0.020344  alpha_Isc=0.004005  IL=5.3624  I0=3.052e-10  nI=0.12439  Rsh=79.3172  Rs=0.081018  BAL=off  Tc=1e-6  Tfilter=5e-5
      settings: SourceProductName=Simscape Electrical
  + : PMIOPort  Side=Right
  - : PMIOPort  Port=2  Side=Right
  wires:
  In2/1 -> PV Module 5/2
  In1/1 -> PV Module 5/1
  connections:
  Diode1/RConn1 -- PV Module 5/RConn1 -- +/RConn1
  PV Module 5/RConn2 -- -/RConn1 -- Diode1/LConn1

== system PSO_BON/Phasor PSO1/Panel Surya/Subsystem2 ==
  In1 : Inport
  In2 : Inport  Port=2
  Diode1 : powerlib/Power Electronics/Diode  Ron=0.001  Lon=0  Vf=0.7  IC=0  UseSnubber=off  Rs=1e5*inf  Cs=inf  Measurements=off
      settings: SourceProductName=Simscape Electrical
  PV Module 5 : re_lib/Solar/PV Array  Npar=1  Nser=1  PlotType=one module @ 25 deg.C & specified irradiances  S_vec="[ 1000  800  100 200]"  Temp_C_vec="[ 45 25  ]"  ModuleName=SunPower SPR-315E-WHT-D  PlotWhenSelected=off  Pm=315.072  Ncell=96  Voc=64.6  Isc=6.14  Vm=54.7  Im=5.76  beta_Voc_pc=-0.27269  alpha_Isc_pc=0.061694  beta_Voc=-0.17616  alpha_Isc=0.003788  IL=6.1461  I0=6.5043e-12  nI=0.9507  Rsh=430.0559  Rs=0.43042  BAL=off  Tc=1e-6  Tfilter=5e-5
      settings: SourceProductName=Simscape Electrical
  + : PMIOPort  Side=Right
  - : PMIOPort  Port=2  Side=Right
  wires:
  In1/1 -> PV Module 5/1
  In2/1 -> PV Module 5/2
  connections:
  Diode1/LConn1 -- -/RConn1 -- PV Module 5/RConn2
  +/RConn1 -- PV Module 5/RConn1 -- Diode1/RConn1

== system PSO_BON/Phasor PSO1/Panel Surya/Subsystem3 ==
  In1 : Inport
  In2 : Inport  Port=2
  Diode1 : powerlib/Power Electronics/Diode  Ron=0.001  Lon=0  Vf=0.7  IC=0  UseSnubber=off  Rs=1e5*inf  Cs=inf  Measurements=off
      settings: SourceProductName=Simscape Electrical
  PV Module 5 : re_lib/Solar/PV Array  Npar=1  Nser=1  PlotType=one module @ 25 deg.C & specified irradiances  S_vec="[ 1000  800  100 200]"  Temp_C_vec="[ 45 25  ]"  ModuleName=SunPower SPR-315E-WHT-D  PlotWhenSelected=off  Pm=315.072  Ncell=96  Voc=64.6  Isc=6.14  Vm=54.7  Im=5.76  beta_Voc_pc=-0.27269  alpha_Isc_pc=0.061694  beta_Voc=-0.17616  alpha_Isc=0.003788  IL=6.1461  I0=6.5043e-12  nI=0.9507  Rsh=430.0559  Rs=0.43042  BAL=off  Tc=1e-6  Tfilter=5e-5
      settings: SourceProductName=Simscape Electrical
  + : PMIOPort  Side=Right
  - : PMIOPort  Port=2  Side=Right
  wires:
  In2/1 -> PV Module 5/2
  In1/1 -> PV Module 5/1
  connections:
  Diode1/RConn1 -- PV Module 5/RConn1 -- +/RConn1
  PV Module 5/RConn2 -- -/RConn1 -- Diode1/LConn1

== system PSO_BON/Phasor PSO1/Panel Surya/Subsystem4 ==
  In1 : Inport
  In2 : Inport  Port=2
  Diode1 : powerlib/Power Electronics/Diode  Ron=0.001  Lon=0  Vf=0.7  IC=0  UseSnubber=off  Rs=1e5*inf  Cs=inf  Measurements=off
      settings: SourceProductName=Simscape Electrical
  PV Module 5 : re_lib/Solar/PV Array  Npar=1  Nser=1  PlotType=one module @ 25 deg.C & specified irradiances  S_vec="[ 1000  800  100 200]"  Temp_C_vec="[ 45 25  ]"  ModuleName=SunPower SPR-315E-WHT-D  PlotWhenSelected=off  Pm=315.072  Ncell=96  Voc=64.6  Isc=6.14  Vm=54.7  Im=5.76  beta_Voc_pc=-0.27269  alpha_Isc_pc=0.061694  beta_Voc=-0.17616  alpha_Isc=0.003788  IL=6.1461  I0=6.5043e-12  nI=0.9507  Rsh=430.0559  Rs=0.43042  BAL=off  Tc=1e-6  Tfilter=1.25e-5
      settings: SourceProductName=Simscape Electrical
  + : PMIOPort  Side=Right
  - : PMIOPort  Port=2  Side=Right
  wires:
  In2/1 -> PV Module 5/2
  In1/1 -> PV Module 5/1
  connections:
  Diode1/RConn1 -- PV Module 5/RConn1 -- +/RConn1
  PV Module 5/RConn2 -- -/RConn1 -- Diode1/LConn1

== system PSO_BON/Phasor PSO1/Panel Surya/Subsystem5 ==
  In1 : Inport
  In2 : Inport  Port=2
  Diode1 : powerlib/Power Electronics/Diode  Ron=0.001  Lon=0  Vf=0.7  IC=0  UseSnubber=off  Rs=1e5*inf  Cs=inf  Measurements=off
      settings: SourceProductName=Simscape Electrical
  PV Module 5 : re_lib/Solar/PV Array  Npar=1  Nser=1  PlotType=one module @ 25 deg.C & specified irradiances  S_vec="[ 1000  800  100 200]"  Temp_C_vec="[ 45 25  ]"  ModuleName=SunPower SPR-315E-WHT-D  PlotWhenSelected=off  Pm=315.072  Ncell=96  Voc=64.6  Isc=6.14  Vm=54.7  Im=5.76  beta_Voc_pc=-0.27269  alpha_Isc_pc=0.061694  beta_Voc=-0.17616  alpha_Isc=0.003788  IL=6.1461  I0=6.5043e-12  nI=0.9507  Rsh=430.0559  Rs=0.43042  BAL=off  Tc=1e-6  Tfilter=1.25e-5
      settings: SourceProductName=Simscape Electrical
  + : PMIOPort  Side=Right
  - : PMIOPort  Port=2  Side=Right
  wires:
  In1/1 -> PV Module 5/1
  In2/1 -> PV Module 5/2
  connections:
  Diode1/LConn1 -- -/RConn1 -- PV Module 5/RConn2
  +/RConn1 -- PV Module 5/RConn1 -- Diode1/RConn1

== system PSO_BON/Phasor PSO1/Panel Surya/Subsystem6 ==
  In1 : Inport
  In2 : Inport  Port=2
  Diode1 : powerlib/Power Electronics/Diode  Ron=0.001  Lon=0  Vf=0.7  IC=0  UseSnubber=off  Rs=1e5*inf  Cs=inf  Measurements=off
      settings: SourceProductName=Simscape Electrical
  PV Module 5 : re_lib/Solar/PV Array  Npar=1  Nser=1  PlotType=one module @ 25 deg.C & specified irradiances  S_vec="[ 1000  800  100 200]"  Temp_C_vec="[ 45 25  ]"  ModuleName=SunPower SPR-315E-WHT-D  PlotWhenSelected=off  Pm=315.072  Ncell=96  Voc=64.6  Isc=6.14  Vm=54.7  Im=5.76  beta_Voc_pc=-0.27269  alpha_Isc_pc=0.061694  beta_Voc=-0.17616  alpha_Isc=0.003788  IL=6.1461  I0=6.5043e-12  nI=0.9507  Rsh=430.0559  Rs=0.43042  BAL=off  Tc=1e-6  Tfilter=1.25e-5
      settings: SourceProductName=Simscape Electrical
  + : PMIOPort  Side=Right
  - : PMIOPort  Port=2  Side=Right
  wires:
  In2/1 -> PV Module 5/2
  In1/1 -> PV Module 5/1
  connections:
  Diode1/RConn1 -- PV Module 5/RConn1 -- +/RConn1
  PV Module 5/RConn2 -- -/RConn1 -- Diode1/LConn1

== system PSO_BON/Phasor PSO1/Panel Surya/Subsystem7 ==
  In1 : Inport
  In2 : Inport  Port=2
  Diode1 : powerlib/Power Electronics/Diode  Ron=0.001  Lon=0  Vf=0.7  IC=0  UseSnubber=off  Rs=1e5*inf  Cs=inf  Measurements=off
      settings: SourceProductName=Simscape Electrical
  PV Module 5 : re_lib/Solar/PV Array  Npar=1  Nser=1  PlotType=one module @ 25 deg.C & specified irradiances  S_vec="[ 1000  800  100 200]"  Temp_C_vec="[ 45 25  ]"  ModuleName=SunPower SPR-315E-WHT-D  PlotWhenSelected=off  Pm=315.072  Ncell=96  Voc=64.6  Isc=6.14  Vm=54.7  Im=5.76  beta_Voc_pc=-0.27269  alpha_Isc_pc=0.061694  beta_Voc=-0.17616  alpha_Isc=0.003788  IL=6.1461  I0=6.5043e-12  nI=0.9507  Rsh=430.0559  Rs=0.43042  BAL=off  Tc=1e-6  Tfilter=1.25e-5
      settings: SourceProductName=Simscape Electrical
  + : PMIOPort  Side=Right
  - : PMIOPort  Port=2  Side=Right
  wires:
  In1/1 -> PV Module 5/1
  In2/1 -> PV Module 5/2
  connections:
  Diode1/LConn1 -- -/RConn1 -- PV Module 5/RConn2
  +/RConn1 -- PV Module 5/RConn1 -- Diode1/RConn1

== system PSO_BON/Phasor PSO1/Panel Surya/Subsystem8 ==
  Gain{,1..3} (4 alike) : Gain  Gain=1000
  Signal Builder : Subsystem  Tag=STV Subsys  LoadFcn=sigbuilder_block('load');  StartFcn=sigbuilder_block('start');  StopFcn=sigbuilder_block('stop');  ClipboardFcn=sigbuilder_block('clipboard');  mask(Sigbuilder block){tuvar=[0:10]}
      mask help: Simulink:masks:SigbuilderBlock_MD
      mask init:
      | if ~strcmp(get_param(bdroot(gcbh),'SimulationStatus'),'stopped') tuvar = sigbuilder_block('maskInit'); end
      settings: CopyFcn=sigbuilder_block('copy');  DeleteFcn=sigbuilder_block('delete');  ModelCloseFcn=sigbuilder_block('modelClose');  PreSaveFcn=sigbuilder_block('preSave');  PauseFcn=sigbuilder_block('pause');  ContinueFcn=sigbuilder_block('continue');  NameChangeFcn=sigbuilder_block('namechange');  OpenFcn=sigbuilder_block('open',[0.75 36.75 510.75 475.5 ]);  CloseFcn=sigbuilder_block('close');
      mask Display: plot(0, 0, 100, 100,[2, 2, 32, 32, 2], [68, 8, 8, 68, 68],[32, 2], [38, 38], [32, 19, 2],[53, 60, 44], [32, 17, 17, 2],[16, 16, 31, 31]);txt = getActiveGroup(gcbh);text(2, 100, txt,'verticalAlignment', 'top');
  Out1 : Outport
  Out2 : Outport  Port=2
  Out3 : Outport  Port=3
  Out4 : Outport  Port=4
  wires:
  Gain/1 -> Out1/1
  Signal Builder/1(Signal 2) -> Gain/1
  Gain1/1 -> Out2/1
  Signal Builder/2(Signal 1) -> Gain1/1
  Gain2/1 -> Out3/1
  Signal Builder/3(Signal 3) -> Gain2/1
  Gain3/1 -> Out4/1
  Signal Builder/4(Signal 4) -> Gain3/1

== system PSO_BON/Phasor PSO1/Panel Surya/Subsystem9 ==
  Gain{,1..3} (4 alike) : Gain  Gain=1000
  Signal Builder : Subsystem  Tag=STV Subsys  LoadFcn=sigbuilder_block('load');  StartFcn=sigbuilder_block('start');  StopFcn=sigbuilder_block('stop');  ClipboardFcn=sigbuilder_block('clipboard');  mask(Sigbuilder block){tuvar=[0:10]}
      mask help: Simulink:masks:SigbuilderBlock_MD
      mask init:
      | if ~strcmp(get_param(bdroot(gcbh),'SimulationStatus'),'stopped') tuvar = sigbuilder_block('maskInit'); end
      settings: CopyFcn=sigbuilder_block('copy');  DeleteFcn=sigbuilder_block('delete');  ModelCloseFcn=sigbuilder_block('modelClose');  PreSaveFcn=sigbuilder_block('preSave');  PauseFcn=sigbuilder_block('pause');  ContinueFcn=sigbuilder_block('continue');  NameChangeFcn=sigbuilder_block('namechange');  OpenFcn=sigbuilder_block('open',[0.75 36.75 510.75 475.5 ]);  CloseFcn=sigbuilder_block('close');
      mask Display: plot(0, 0, 100, 100,[2, 2, 32, 32, 2], [68, 8, 8, 68, 68],[32, 2], [38, 38], [32, 19, 2],[53, 60, 44], [32, 17, 17, 2],[16, 16, 31, 31]);txt = getActiveGroup(gcbh);text(2, 100, txt,'verticalAlignment', 'top');
  Out1 : Outport
  Out2 : Outport  Port=2
  Out3 : Outport  Port=3
  Out4 : Outport  Port=4
  wires:
  Signal Builder/4(Signal 4) -> Gain3/1
  Gain3/1 -> Out4/1
  Signal Builder/3(Signal 3) -> Gain2/1
  Gain2/1 -> Out3/1
  Signal Builder/2(Signal 1) -> Gain1/1
  Gain1/1 -> Out2/1
  Signal Builder/1(Signal 2) -> Gain/1
  Gain/1 -> Out1/1

== system PSO_BON/Phasor PSO1/Panel Surya2/Subsystem ==
  In1 : Inport
  In2 : Inport  Port=2
  Diode1 : powerlib/Power Electronics/Diode  Ron=0.001  Lon=0  Vf=0.7  IC=0  UseSnubber=off  Rs=1e5*inf  Cs=inf  Measurements=off
      settings: SourceProductName=Simscape Electrical
  PV Module 5 : re_lib/Solar/PV Array  Npar=1  Nser=1  PlotType=one module @ 25 deg.C & specified irradiances  S_vec="[ 1000  800  100 200]"  Temp_C_vec="[ 45 25  ]"  ModuleName=SunPower SPR-315E-WHT-D  PlotWhenSelected=off  Pm=315.072  Ncell=96  Voc=64.6  Isc=6.14  Vm=54.7  Im=5.76  beta_Voc_pc=-0.27269  alpha_Isc_pc=0.061694  beta_Voc=-0.17616  alpha_Isc=0.003788  IL=6.1461  I0=6.5043e-12  nI=0.9507  Rsh=430.0559  Rs=0.43042  BAL=off  Tc=1e-6  Tfilter=5e-5
      settings: SourceProductName=Simscape Electrical
  + : PMIOPort  Side=Right
  - : PMIOPort  Port=2  Side=Right
  wires:
  In1/1 -> PV Module 5/1
  In2/1 -> PV Module 5/2
  connections:
  Diode1/LConn1 -- -/RConn1 -- PV Module 5/RConn2
  +/RConn1 -- PV Module 5/RConn1 -- Diode1/RConn1

== system PSO_BON/Phasor PSO1/Panel Surya2/Subsystem1 ==
  In1 : Inport
  In2 : Inport  Port=2
  Diode1 : powerlib/Power Electronics/Diode  Ron=0.001  Lon=0  Vf=0.7  IC=0  UseSnubber=off  Rs=1e5*inf  Cs=inf  Measurements=off
      settings: SourceProductName=Simscape Electrical
  PV Module 5 : re_lib/Solar/PV Array  Npar=1  Nser=1  PlotType=one module @ 25 deg.C & specified irradiances  S_vec="[ 1000  800  100 200]"  Temp_C_vec="[ 45 25  ]"  ModuleName=SunPower SPR-315E-WHT-D  PlotWhenSelected=off  Pm=315.072  Ncell=96  Voc=64.6  Isc=6.14  Vm=54.7  Im=5.76  beta_Voc_pc=-0.27269  alpha_Isc_pc=0.061694  beta_Voc=-0.17616  alpha_Isc=0.003788  IL=6.1461  I0=6.5043e-12  nI=0.9507  Rsh=430.0559  Rs=0.43042  BAL=off  Tc=1e-6  Tfilter=5e-5
      settings: SourceProductName=Simscape Electrical
  + : PMIOPort  Side=Right
  - : PMIOPort  Port=2  Side=Right
  wires:
  In2/1 -> PV Module 5/2
  In1/1 -> PV Module 5/1
  connections:
  Diode1/RConn1 -- PV Module 5/RConn1 -- +/RConn1
  PV Module 5/RConn2 -- -/RConn1 -- Diode1/LConn1

== system PSO_BON/Phasor PSO1/Panel Surya2/Subsystem10 ==
  Gain : Gain  Gain=1000
  Signal Builder : Subsystem  Tag=STV Subsys  LoadFcn=sigbuilder_block('load');  StartFcn=sigbuilder_block('start');  StopFcn=sigbuilder_block('stop');  ClipboardFcn=sigbuilder_block('clipboard');  mask(Sigbuilder block){tuvar=[0:10]}
      mask help: Simulink:masks:SigbuilderBlock_MD
      mask init:
      | if ~strcmp(get_param(bdroot(gcbh),'SimulationStatus'),'stopped') tuvar = sigbuilder_block('maskInit'); end
      settings: CopyFcn=sigbuilder_block('copy');  DeleteFcn=sigbuilder_block('delete');  ModelCloseFcn=sigbuilder_block('modelClose');  PreSaveFcn=sigbuilder_block('preSave');  PauseFcn=sigbuilder_block('pause');  ContinueFcn=sigbuilder_block('continue');  NameChangeFcn=sigbuilder_block('namechange');  OpenFcn=sigbuilder_block('open',[367.8 96.6 550.8 400.2 ]);  CloseFcn=sigbuilder_block('close');
      mask Display: plot(0, 0, 100, 100,[2, 2, 32, 32, 2], [68, 8, 8, 68, 68],[32, 2], [38, 38], [32, 19, 2],[53, 60, 44], [32, 17, 17, 2],[16, 16, 31, 31]);txt = getActiveGroup(gcbh);text(2, 100, txt,'verticalAlignment', 'top');
  Out1 : Outport
  wires:
  Signal Builder/1(Signal 2) -> Gain/1
  Gain/1 -> Out1/1

== system PSO_BON/Phasor PSO1/Panel Surya2/Subsystem11 ==
  Gain : Gain  Gain=1000
  Signal Builder : Subsystem  Tag=STV Subsys  LoadFcn=sigbuilder_block('load');  StartFcn=sigbuilder_block('start');  StopFcn=sigbuilder_block('stop');  ClipboardFcn=sigbuilder_block('clipboard');  mask(Sigbuilder block){tuvar=[0:10]}
      mask help: Simulink:masks:SigbuilderBlock_MD
      mask init:
      | if ~strcmp(get_param(bdroot(gcbh),'SimulationStatus'),'stopped') tuvar = sigbuilder_block('maskInit'); end
      settings: CopyFcn=sigbuilder_block('copy');  DeleteFcn=sigbuilder_block('delete');  ModelCloseFcn=sigbuilder_block('modelClose');  PreSaveFcn=sigbuilder_block('preSave');  PauseFcn=sigbuilder_block('pause');  ContinueFcn=sigbuilder_block('continue');  NameChangeFcn=sigbuilder_block('namechange');  OpenFcn=sigbuilder_block('open',[367.8 96.6 550.8 400.2 ]);  CloseFcn=sigbuilder_block('close');
      mask Display: plot(0, 0, 100, 100,[2, 2, 32, 32, 2], [68, 8, 8, 68, 68],[32, 2], [38, 38], [32, 19, 2],[53, 60, 44], [32, 17, 17, 2],[16, 16, 31, 31]);txt = getActiveGroup(gcbh);text(2, 100, txt,'verticalAlignment', 'top');
  Out1 : Outport
  wires:
  Gain/1 -> Out1/1
  Signal Builder/1(Signal 2) -> Gain/1

== system PSO_BON/Phasor PSO1/Panel Surya2/Subsystem2 ==
  In1 : Inport
  In2 : Inport  Port=2
  Diode1 : powerlib/Power Electronics/Diode  Ron=0.001  Lon=0  Vf=0.7  IC=0  UseSnubber=off  Rs=1e5*inf  Cs=inf  Measurements=off
      settings: SourceProductName=Simscape Electrical
  PV Module 5 : re_lib/Solar/PV Array  Npar=1  Nser=1  PlotType=one module @ 25 deg.C & specified irradiances  S_vec="[ 1000  800  100 200]"  Temp_C_vec="[ 45 25  ]"  ModuleName=SunPower SPR-315E-WHT-D  PlotWhenSelected=off  Pm=315.072  Ncell=96  Voc=64.6  Isc=6.14  Vm=54.7  Im=5.76  beta_Voc_pc=-0.27269  alpha_Isc_pc=0.061694  beta_Voc=-0.17616  alpha_Isc=0.003788  IL=6.1461  I0=6.5043e-12  nI=0.9507  Rsh=430.0559  Rs=0.43042  BAL=off  Tc=1e-6  Tfilter=5e-5
      settings: SourceProductName=Simscape Electrical
  + : PMIOPort  Side=Right
  - : PMIOPort  Port=2  Side=Right
  wires:
  In1/1 -> PV Module 5/1
  In2/1 -> PV Module 5/2
  connections:
  Diode1/LConn1 -- -/RConn1 -- PV Module 5/RConn2
  +/RConn1 -- PV Module 5/RConn1 -- Diode1/RConn1

== system PSO_BON/Phasor PSO1/Panel Surya2/Subsystem3 ==
  In1 : Inport
  In2 : Inport  Port=2
  Diode1 : powerlib/Power Electronics/Diode  Ron=0.001  Lon=0  Vf=0.7  IC=0  UseSnubber=off  Rs=1e5*inf  Cs=inf  Measurements=off
      settings: SourceProductName=Simscape Electrical
  PV Module 5 : re_lib/Solar/PV Array  Npar=1  Nser=1  PlotType=one module @ 25 deg.C & specified irradiances  S_vec="[ 1000  800  100 200]"  Temp_C_vec="[ 45 25  ]"  ModuleName=SunPower SPR-315E-WHT-D  PlotWhenSelected=off  Pm=315.072  Ncell=96  Voc=64.6  Isc=6.14  Vm=54.7  Im=5.76  beta_Voc_pc=-0.27269  alpha_Isc_pc=0.061694  beta_Voc=-0.17616  alpha_Isc=0.003788  IL=6.1461  I0=6.5043e-12  nI=0.9507  Rsh=430.0559  Rs=0.43042  BAL=off  Tc=1e-6  Tfilter=5e-5
      settings: SourceProductName=Simscape Electrical
  + : PMIOPort  Side=Right
  - : PMIOPort  Port=2  Side=Right
  wires:
  In2/1 -> PV Module 5/2
  In1/1 -> PV Module 5/1
  connections:
  Diode1/RConn1 -- PV Module 5/RConn1 -- +/RConn1
  PV Module 5/RConn2 -- -/RConn1 -- Diode1/LConn1

== system PSO_BON/Phasor PSO1/Panel Surya2/Subsystem4 ==
  In1 : Inport
  In2 : Inport  Port=2
  Diode1 : powerlib/Power Electronics/Diode  Ron=0.001  Lon=0  Vf=0.7  IC=0  UseSnubber=off  Rs=1e5*inf  Cs=inf  Measurements=off
      settings: SourceProductName=Simscape Electrical
  PV Module 5 : re_lib/Solar/PV Array  Npar=1  Nser=1  PlotType=one module @ 25 deg.C & specified irradiances  S_vec="[ 1000  800  100 200]"  Temp_C_vec="[ 45 25  ]"  ModuleName=SunPower SPR-315E-WHT-D  PlotWhenSelected=off  Pm=315.072  Ncell=96  Voc=64.6  Isc=6.14  Vm=54.7  Im=5.76  beta_Voc_pc=-0.27269  alpha_Isc_pc=0.061694  beta_Voc=-0.17616  alpha_Isc=0.003788  IL=6.1461  I0=6.5043e-12  nI=0.9507  Rsh=430.0559  Rs=0.43042  BAL=off  Tc=1e-6  Tfilter=1.25e-5
      settings: SourceProductName=Simscape Electrical
  + : PMIOPort  Side=Right
  - : PMIOPort  Port=2  Side=Right
  wires:
  In2/1 -> PV Module 5/2
  In1/1 -> PV Module 5/1
  connections:
  Diode1/RConn1 -- PV Module 5/RConn1 -- +/RConn1
  PV Module 5/RConn2 -- -/RConn1 -- Diode1/LConn1
